simulink model "sm_DDPG_Training_Circuit"  (R2025b)
settings: Solver=VariableStepAuto  StartTime=0.0  StopTime=2000  RelTol=1e-3
values from neighbouring files (symbols this model uses):
  fD = 3.5243/2    (= 1.76215)    [code_DDPG_Training.m]    (also in code_Experimental_Setup.m; code_SA_TF_Estimator.m = 3.5243)
  fS = 8.4000/2    (= 4.2)    [code_DDPG_Training.m]    (also in code_Experimental_Setup.m; code_SA_TF_Estimator.m = 8.4)
  TIME_DELAY = 2.5/2    (= 1.25)    [code_DDPG_Training.m]    (also in code_Experimental_Setup.m; code_SA_TF_Estimator.m = 2.5)
  Ts = 1.0    (= 1)    [code_DDPG_Training.m]    (also in code_Experimental_Setup.m; code_SA_TF_Estimator.m)
undefined symbols (not defined in the file or in its folder): DiscIntNeverNeededParam
libraries: simulink x2, rllib x1
settings Model: Creator=rajeshs  LastModifiedBy=kinki
settings SolverCC: AlgebraicLoopSolver=TrustRegion
settings DebuggingCC: UnconnectedInputMsg=warning  UnconnectedOutputMsg=warning  UnconnectedLineMsg=warning
settings ModelReferenceCC: EnableRefExpFcnMdlSchedulingChecks=on
settings SFSimCC: CustomCodeUndefinedFunction=UseInterfaceOnly
settings RTWCC: GPUComputeCapability=3.5  DLArmComputeVersion=19.05
settings SimscapeCC: SimscapeLogDataHistory=5000  SimscapeLogDecimation=1

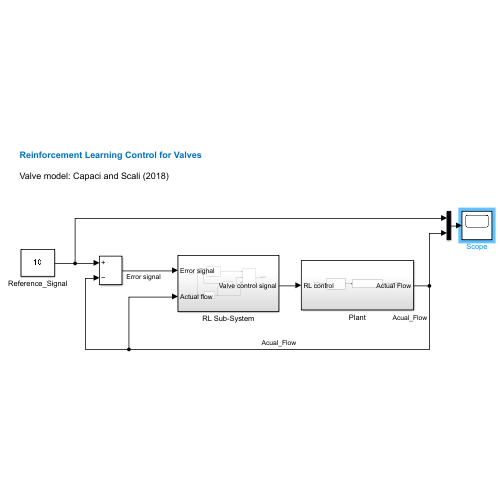
[thumbnail: Simulink's stored preview of the top-level diagram]
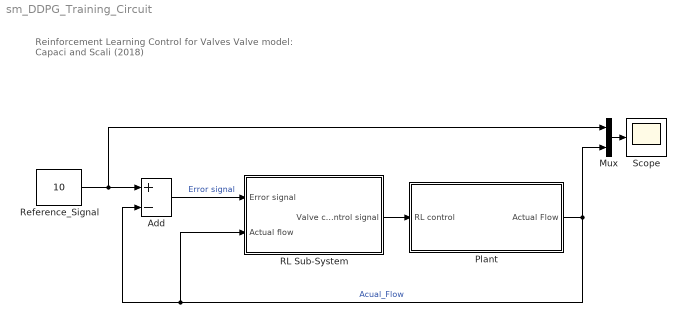
== system sm_DDPG_Training_Circuit ==
  note: Reinforcement Learning Control for Valves
      |
      | Valve model: Capaci and Scali (2018)
  Add : Sum  Inputs=+-
  Mux : Mux  Inputs=2
  Plant : Subsystem
  RL Sub-System : Subsystem
  Reference_Signal : Constant  Value=10
  Scope : Scope
      settings: ActiveDisplayYMinimum=-1  ActiveDisplayYMaximum=110  YLabel=Controlled vs Ref. Flow
  wires:
  Mux/1 -> Scope/1
  Add/1 -> RL Sub-System/1(Error signal)  "Error signal"
  Plant/1(Actual Flow) -> Add/2, RL Sub-System/2(Actual flow), Mux/2  "Acual_Flow"
  Reference_Signal/1 -> Mux/1, Add/1
  RL Sub-System/1(Valve control signal) -> Plant/1(RL control)

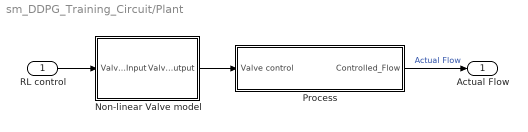
== system sm_DDPG_Training_Circuit/Plant ==
  RL control : Inport
  Non-linear Valve model : Subsystem
  Process : Subsystem
  Actual Flow : Outport  VectorParamsAs1DForOutWhenUnconnected=off
  wires:
  Non-linear Valve model/1(ValveOutput) -> Process/1(Valve control)
  Process/1(Controlled_Flow) -> Actual Flow/1  "Actual Flow"
  RL control/1 -> Non-linear Valve model/1(ValveInput)

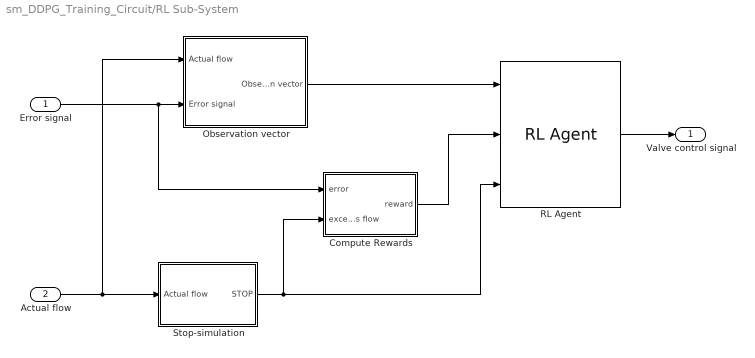
== system sm_DDPG_Training_Circuit/RL Sub-System ==
  Error signal : Inport
  Actual flow : Inport  Port=2
  Compute Rewards : Subsystem
  Observation vector : Subsystem
  RL Agent : rllib/RL Agent  Agent=agent  ExternalActionAsInput=off  ProvideLastAction=off  ProvideCumRwd=off  TreatAsDirectFeedthrough=on  UseStrictObservationDataTypes=off
  Stop-simulation : Subsystem
  Valve control signal : Outport  VectorParamsAs1DForOutWhenUnconnected=off
  wires:
  Stop-simulation/1(STOP) -> RL Agent/3, Compute Rewards/2(exceeds flow)
  Error signal/1 -> Compute Rewards/1(error), Observation vector/2(Error signal)
  Compute Rewards/1(reward) -> RL Agent/2
  Observation vector/1(Observation vector) -> RL Agent/1
  RL Agent/1 -> Valve control signal/1
  Actual flow/1 -> Observation vector/1(Actual flow), Stop-simulation/1(Actual flow)

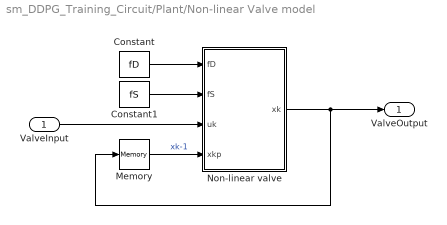
== system sm_DDPG_Training_Circuit/Plant/Non-linear Valve model ==
  ValveInput : Inport
  Constant : Constant  Value=fD
  Constant1 : Constant  Value=fS
  Memory : Memory
  Non-linear valve : MATLAB Function  TreatAsAtomicUnit=on
  ValveOutput : Outport  VectorParamsAs1DForOutWhenUnconnected=off
  wires:
  Non-linear valve/1(xk) -> ValveOutput/1, Memory/1
  Memory/1 -> Non-linear valve/4(xkp)  "xk-1"
  ValveInput/1 -> Non-linear valve/3(uk)
  Constant/1 -> Non-linear valve/1(fD)
  Constant1/1 -> Non-linear valve/2(fS)

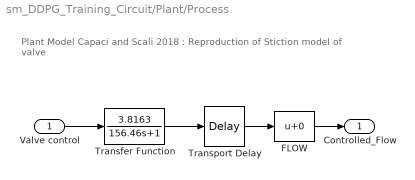
== system sm_DDPG_Training_Circuit/Plant/Process ==
  note: Plant Model
      |
      | Capaci and Scali 2018 : Reproduction of Stiction model of valve
  Valve control : Inport
  FLOW : Bias  SaturateOnIntegerOverflow=off
  Transfer Function : TransferFcn  Numerator=[3.8163]  Denominator=[156.46 1]
  "Transport Delay " : TransportDelay  DelayTime=TIME_DELAY
  Controlled_Flow : Outport  VectorParamsAs1DForOutWhenUnconnected=off
  wires:
  FLOW/1 -> Controlled_Flow/1
  Transfer Function/1 -> "Transport Delay "/1
  Valve control/1 -> Transfer Function/1
  "Transport Delay "/1 -> FLOW/1

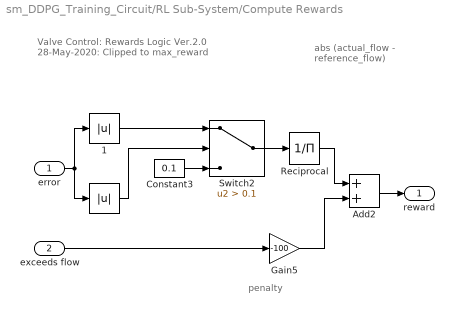
== system sm_DDPG_Training_Circuit/RL Sub-System/Compute Rewards ==
  note: penalty
  note: abs (actual_flow - reference_flow)
  note: Valve Control: Rewards Logic
      | Ver.2.0 28-May-2020: Clipped to max_reward
  error : Inport
  exceeds flow : Inport  Port=2
  " " : Abs  SaturateOnIntegerOverflow=off
  " 1" : Abs  SaturateOnIntegerOverflow=off
  Add2 : Sum
  Constant3 : Constant  Value=0.1
  Gain5 : Gain  Gain=-100
  Reciprocal : Product  Inputs=/
  Switch2 : Switch  Criteria=u2 > Threshold  Threshold=0.1  SaturateOnIntegerOverflow=off  InputSameDT=off
  reward : Outport  VectorParamsAs1DForOutWhenUnconnected=off
  wires:
  Gain5/1 -> Add2/2
  exceeds flow/1 -> Gain5/1
  error/1 -> " 1"/1, " "/1
  Add2/1 -> reward/1
  " "/1 -> Switch2/2
  Reciprocal/1 -> Add2/1
  " 1"/1 -> Switch2/1
  Switch2/1 -> Reciprocal/1
  Constant3/1 -> Switch2/3

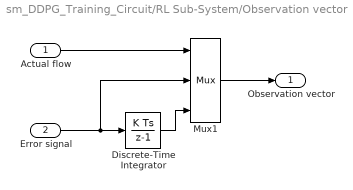
== system sm_DDPG_Training_Circuit/RL Sub-System/Observation vector ==
  Actual flow : Inport
  Error signal : Inport  Port=2
  Discrete-Time Integrator : DiscreteIntegrator  SampleTime=Ts  ICPrevOutput=DiscIntNeverNeededParam  ICPrevScaledInput=DiscIntNeverNeededParam
  Mux1 : Mux  Inputs=3
  Observation vector : Outport  VectorParamsAs1DForOutWhenUnconnected=off
  wires:
  Discrete-Time Integrator/1 -> Mux1/3
  Mux1/1 -> Observation vector/1
  Error signal/1 -> Discrete-Time Integrator/1, Mux1/2
  Actual flow/1 -> Mux1/1

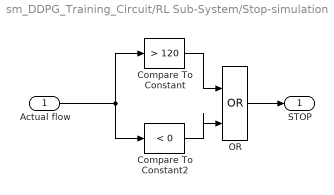
== system sm_DDPG_Training_Circuit/RL Sub-System/Stop-simulation ==
  Actual flow : Inport
  Compare To Constant : simulink/Logic and Bit Operations/Compare To Constant  relop=>  const=120  OutDataTypeStr=boolean
  Compare To Constant2 : simulink/Logic and Bit Operations/Compare To Constant  relop=<  const=0  OutDataTypeStr=boolean
  OR : Logic  Operator=OR  IconShape=distinctive  AllPortsSameDT=off  OutDataTypeStr=boolean
  STOP : Outport  VectorParamsAs1DForOutWhenUnconnected=off
  wires:
  Compare To Constant/1 -> OR/1
  Actual flow/1 -> Compare To Constant/1, Compare To Constant2/1
  Compare To Constant2/1 -> OR/2
  OR/1 -> STOP/1

== matlab function sm_DDPG_Training_Circuit/Plant/Non-linear Valve model/Non-linear valve ==
  data: fD input; fS input; uk input; xk output; xkp input
function xk = fcn(fD, fS, uk, xkp)
% -------------------------------------------------------------------------
% TRAINING circuit for DDPG-RL Agent | Plant Model (RLVC4 | 09-Oct-2020)
% Non-Linear valve model: Capaci and Scali (2018)
% -------------------------------------------------------------------------
% uk - fD   if uk - xk−1 > fS
% uk + fD   if uk - xk−1 < -fS
% xk - 1    if |uk - xk−1| < fS
% -------------------------------------------------------------------------
% Graded Learning Stages:
% GRADE_I    TIME_DELAY=0.1; fS = 8.4/10; fD = 3.5243/10 
% GRADE_II   TIME_DELAY=0.5; fS = 8.4/5; fD = 3.5243/5
% GRADE_III  TIME_DELAY=1.5; fS = 8.4/2; fD = 3.5243/2
% GRADE_IV   TIME_DELAY=1.5; fS = 8.4/1.5; fD = 3.5243/1.5
% GRADE_IV   TIME_DELAY=1.5, fS/1.5 and fD/1.5
% GRADE_V    TIME_DELAY=2.0, fS/1.5 and fD/1.5
% GRADE_VI   TIME_DELAY=2.5, fS/1.0 and fD/1.0
% -------------------------------------------------------------------------
    
    % For PPO, the action is a column vector [2 1], therefore we need
    %  to convert it to a [1 1]. reshape can't be used because Reshape
    %  needs to retain number of elements. Manually extract first value
    % PPO action output is (1) Mean (2) Std. Dev and therefore we need only
    % the first value
    uk = uk(1,1);
     
    t_xk = 0.0;
   
    if ((uk-xkp) > fS)
        t_xk = uk - fD;
    elseif ((uk-xkp) < -1*fS)
        t_xk = uk + fD;
    elseif (abs(uk-xkp) < fS)
        t_xk = xkp;
    end
    
xk = t_xk;
